simulink model "IEEE33_2018"  (R2018b)
settings: Solver=VariableStepAuto  StartTime=0.0  StopTime=0.04  RelTol=1e-3
undefined symbols (not defined in the file or in its folder): D11, Delta
libraries: powerlib x134
settings Model: Creator=zyx  LastModifiedBy=zyx53
settings DataIOCC: ReturnWorkspaceOutputs=on
settings DebuggingCC: UnconnectedInputMsg=none  UnconnectedOutputMsg=none  UnconnectedLineMsg=none
settings ModelReferenceCC: EnableRefExpFcnMdlSchedulingChecks=off
settings RTWCC: Description=Generic Real-Time Target

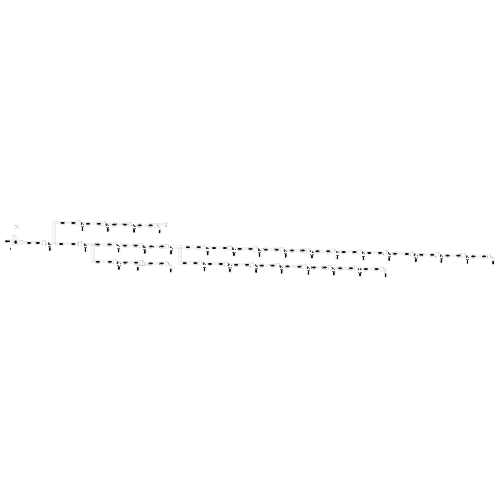
[thumbnail: Simulink's stored preview of the top-level diagram]
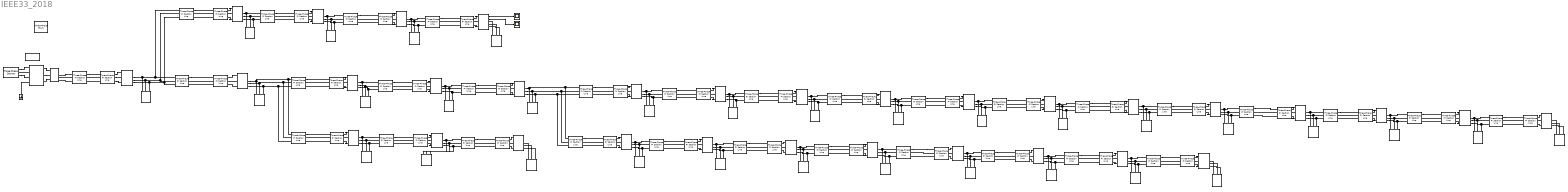
== system IEEE33_2018 ==
  Ground : powerlib/Elements/Ground  LConnTagsString=a
  Node1 : powerlib/Elements/Three-Phase Series RLC Load  LConnTagsString=A|B|C  Configuration=Y (grounded)  NominalVoltage=10.5e3  Vabc=[1e3 1e3 1e3]  Vabcp=[1e3 1e3 1e3]  NominalFrequency=50  UnbalancedPower=off  ActivePower=1636286.9  InductivePower=425428.22  CapacitivePower=0  Pabc=[10e3 9e3 11e3]  QLabc=[100 90 110]  QCabc=[100 90 110]  Pabcp=[10e3 9e3 11e3]  QLabcp=[100 90 110]  QCabcp=[100 90 110]  Measurements=None  LoadType=constant Z
  Node10 : powerlib/Elements/Three-Phase Series RLC Load  LConnTagsString=A|B|C  Configuration=Y (grounded)  NominalVoltage=10.5e3  Vabc=[1e3 1e3 1e3]  Vabcp=[1e3 1e3 1e3]  NominalFrequency=50  UnbalancedPower=off  ActivePower=1452178.34  InductivePower=456782.16  CapacitivePower=0  Pabc=[10e3 9e3 11e3]  QLabc=[100 90 110]  QCabc=[100 90 110]  Pabcp=[10e3 9e3 11e3]  QLabcp=[100 90 110]  QCabcp=[100 90 110]  Measurements=None  LoadType=constant Z
  Node11 : powerlib/Elements/Three-Phase Series RLC Load  LConnTagsString=A|B|C  Configuration=Y (grounded)  NominalVoltage=10.5e3  Vabc=[1e3 1e3 1e3]  Vabcp=[1e3 1e3 1e3]  NominalFrequency=50  UnbalancedPower=off  ActivePower=1330341.72  InductivePower=405395.01  CapacitivePower=0  Pabc=[10e3 9e3 11e3]  QLabc=[100 90 110]  QCabc=[100 90 110]  Pabcp=[10e3 9e3 11e3]  QLabcp=[100 90 110]  QCabcp=[100 90 110]  Measurements=None  LoadType=constant Z
  Node12 : powerlib/Elements/Three-Phase Series RLC Load  LConnTagsString=A|B|C  Configuration=Y (grounded)  NominalVoltage=10.5e3  Vabc=[1e3 1e3 1e3]  Vabcp=[1e3 1e3 1e3]  NominalFrequency=50  UnbalancedPower=off  ActivePower=1512319.02  InductivePower=477916.72  CapacitivePower=0  Pabc=[10e3 9e3 11e3]  QLabc=[100 90 110]  QCabc=[100 90 110]  Pabcp=[10e3 9e3 11e3]  QLabcp=[100 90 110]  QCabcp=[100 90 110]  Measurements=None  LoadType=constant Z
  Node13 : powerlib/Elements/Three-Phase Series RLC Load  LConnTagsString=A|B|C  Configuration=Y (grounded)  NominalVoltage=10.5e3  Vabc=[1e3 1e3 1e3]  Vabcp=[1e3 1e3 1e3]  NominalFrequency=50  UnbalancedPower=off  ActivePower=1673604.27  InductivePower=412990.62  CapacitivePower=0  Pabc=[10e3 9e3 11e3]  QLabc=[100 90 110]  QCabc=[100 90 110]  Pabcp=[10e3 9e3 11e3]  QLabcp=[100 90 110]  QCabcp=[100 90 110]  Measurements=None  LoadType=constant Z
  Node14 : powerlib/Elements/Three-Phase Series RLC Load  LConnTagsString=A|B|C  Configuration=Y (grounded)  NominalVoltage=10.5e3  Vabc=[1e3 1e3 1e3]  Vabcp=[1e3 1e3 1e3]  NominalFrequency=50  UnbalancedPower=off  ActivePower=1527529.46  InductivePower=446939.06  CapacitivePower=0  Pabc=[10e3 9e3 11e3]  QLabc=[100 90 110]  QCabc=[100 90 110]  Pabcp=[10e3 9e3 11e3]  QLabcp=[100 90 110]  QCabcp=[100 90 110]  Measurements=None  LoadType=constant Z
  Node15 : powerlib/Elements/Three-Phase Series RLC Load  LConnTagsString=A|B|C  Configuration=Y (grounded)  NominalVoltage=10.5e3  Vabc=[1e3 1e3 1e3]  Vabcp=[1e3 1e3 1e3]  NominalFrequency=50  UnbalancedPower=off  ActivePower=1304760.83  InductivePower=433712.26  CapacitivePower=0  Pabc=[10e3 9e3 11e3]  QLabc=[100 90 110]  QCabc=[100 90 110]  Pabcp=[10e3 9e3 11e3]  QLabcp=[100 90 110]  QCabcp=[100 90 110]  Measurements=None  LoadType=constant Z
  Node16 : powerlib/Elements/Three-Phase Series RLC Load  LConnTagsString=A|B|C  Configuration=Y (grounded)  NominalVoltage=10.5e3  Vabc=[1e3 1e3 1e3]  Vabcp=[1e3 1e3 1e3]  NominalFrequency=50  UnbalancedPower=off  ActivePower=1364872.92  InductivePower=479428.45  CapacitivePower=0  Pabc=[10e3 9e3 11e3]  QLabc=[100 90 110]  QCabc=[100 90 110]  Pabcp=[10e3 9e3 11e3]  QLabcp=[100 90 110]  QCabcp=[100 90 110]  Measurements=None  LoadType=constant Z
  Node17 : powerlib/Elements/Three-Phase Series RLC Load  LConnTagsString=A|B|C  Configuration=Y (grounded)  NominalVoltage=10.5e3  Vabc=[1e3 1e3 1e3]  Vabcp=[1e3 1e3 1e3]  NominalFrequency=50  UnbalancedPower=off  ActivePower=1424486.02  InductivePower=452853.31  CapacitivePower=0  Pabc=[10e3 9e3 11e3]  QLabc=[100 90 110]  QCabc=[100 90 110]  Pabcp=[10e3 9e3 11e3]  QLabcp=[100 90 110]  QCabcp=[100 90 110]  Measurements=None  LoadType=constant Z
  Node18 : powerlib/Elements/Three-Phase Series RLC Load  LConnTagsString=A|B|C  Configuration=Y (grounded)  NominalVoltage=10.5e3  Vabc=[1e3 1e3 1e3]  Vabcp=[1e3 1e3 1e3]  NominalFrequency=50  UnbalancedPower=off  ActivePower=1366259.49  InductivePower=460198.19  CapacitivePower=0  Pabc=[10e3 9e3 11e3]  QLabc=[100 90 110]  QCabc=[100 90 110]  Pabcp=[10e3 9e3 11e3]  QLabcp=[100 90 110]  QCabcp=[100 90 110]  Measurements=None  LoadType=constant Z
  Node19 : powerlib/Elements/Three-Phase Series RLC Load  LConnTagsString=A|B|C  Configuration=Y (grounded)  NominalVoltage=10.5e3  Vabc=[1e3 1e3 1e3]  Vabcp=[1e3 1e3 1e3]  NominalFrequency=50  UnbalancedPower=off  ActivePower=1405188.51  InductivePower=465407.91  CapacitivePower=0  Pabc=[10e3 9e3 11e3]  QLabc=[100 90 110]  QCabc=[100 90 110]  Pabcp=[10e3 9e3 11e3]  QLabcp=[100 90 110]  QCabcp=[100 90 110]  Measurements=None  LoadType=constant Z
  Node2 : powerlib/Elements/Three-Phase Series RLC Load  LConnTagsString=A|B|C  Configuration=Y (grounded)  NominalVoltage=10.5e3  Vabc=[1e3 1e3 1e3]  Vabcp=[1e3 1e3 1e3]  NominalFrequency=50  UnbalancedPower=off  ActivePower=1625713.93  InductivePower=424352.5  CapacitivePower=0  Pabc=[10e3 9e3 11e3]  QLabc=[100 90 110]  QCabc=[100 90 110]  Pabcp=[10e3 9e3 11e3]  QLabcp=[100 90 110]  QCabcp=[100 90 110]  Measurements=None  LoadType=constant Z
  Node20 : powerlib/Elements/Three-Phase Series RLC Load  LConnTagsString=A|B|C  Configuration=Y (grounded)  NominalVoltage=10.5e3  Vabc=[1e3 1e3 1e3]  Vabcp=[1e3 1e3 1e3]  NominalFrequency=50  UnbalancedPower=off  ActivePower=1575685.8  InductivePower=474815.16  CapacitivePower=0  Pabc=[10e3 9e3 11e3]  QLabc=[100 90 110]  QCabc=[100 90 110]  Pabcp=[10e3 9e3 11e3]  QLabcp=[100 90 110]  QCabcp=[100 90 110]  Measurements=None  LoadType=constant Z
  Node21 : powerlib/Elements/Three-Phase Series RLC Load  LConnTagsString=A|B|C  Configuration=Y (grounded)  NominalVoltage=10.5e3  Vabc=[1e3 1e3 1e3]  Vabcp=[1e3 1e3 1e3]  NominalFrequency=50  UnbalancedPower=off  ActivePower=1480216.64  InductivePower=408382.14  CapacitivePower=0  Pabc=[10e3 9e3 11e3]  QLabc=[100 90 110]  QCabc=[100 90 110]  Pabcp=[10e3 9e3 11e3]  QLabcp=[100 90 110]  QCabcp=[100 90 110]  Measurements=None  LoadType=constant Z
  Node22 : powerlib/Elements/Three-Phase Series RLC Load  LConnTagsString=A|B|C  Configuration=Y (grounded)  NominalVoltage=10.5e3  Vabc=[1e3 1e3 1e3]  Vabcp=[1e3 1e3 1e3]  NominalFrequency=50  UnbalancedPower=off  ActivePower=1391590.79  InductivePower=491333.74  CapacitivePower=0  Pabc=[10e3 9e3 11e3]  QLabc=[100 90 110]  QCabc=[100 90 110]  Pabcp=[10e3 9e3 11e3]  QLabcp=[100 90 110]  QCabcp=[100 90 110]  Measurements=None  LoadType=constant Z
  Node23 : powerlib/Elements/Three-Phase Series RLC Load  LConnTagsString=A|B|C  Configuration=Y (grounded)  NominalVoltage=10.5e3  Vabc=[1e3 1e3 1e3]  Vabcp=[1e3 1e3 1e3]  NominalFrequency=50  UnbalancedPower=off  ActivePower=1360951.21  InductivePower=482581.7  CapacitivePower=0  Pabc=[10e3 9e3 11e3]  QLabc=[100 90 110]  QCabc=[100 90 110]  Pabcp=[10e3 9e3 11e3]  QLabcp=[100 90 110]  QCabcp=[100 90 110]  Measurements=None  LoadType=constant Z
  Node24 : powerlib/Elements/Three-Phase Series RLC Load  LConnTagsString=A|B|C  Configuration=Y (grounded)  NominalVoltage=10.5e3  Vabc=[1e3 1e3 1e3]  Vabcp=[1e3 1e3 1e3]  NominalFrequency=50  UnbalancedPower=off  ActivePower=1515336.97  InductivePower=499613.47  CapacitivePower=0  Pabc=[10e3 9e3 11e3]  QLabc=[100 90 110]  QCabc=[100 90 110]  Pabcp=[10e3 9e3 11e3]  QLabcp=[100 90 110]  QCabcp=[100 90 110]  Measurements=None  LoadType=constant Z
  Node25 : powerlib/Elements/Three-Phase Series RLC Load  LConnTagsString=A|B|C  Configuration=Y (grounded)  NominalVoltage=10.5e3  Vabc=[1e3 1e3 1e3]  Vabcp=[1e3 1e3 1e3]  NominalFrequency=50  UnbalancedPower=off  ActivePower=1331270.21  InductivePower=444267.83  CapacitivePower=0  Pabc=[10e3 9e3 11e3]  QLabc=[100 90 110]  QCabc=[100 90 110]  Pabcp=[10e3 9e3 11e3]  QLabcp=[100 90 110]  QCabcp=[100 90 110]  Measurements=None  LoadType=constant Z
  Node26 : powerlib/Elements/Three-Phase Series RLC Load  LConnTagsString=A|B|C  Configuration=Y (grounded)  NominalVoltage=10.5e3  Vabc=[1e3 1e3 1e3]  Vabcp=[1e3 1e3 1e3]  NominalFrequency=50  UnbalancedPower=off  ActivePower=1342661.11  InductivePower=496189.81  CapacitivePower=0  Pabc=[10e3 9e3 11e3]  QLabc=[100 90 110]  QCabc=[100 90 110]  Pabcp=[10e3 9e3 11e3]  QLabcp=[100 90 110]  QCabcp=[100 90 110]  Measurements=None  LoadType=constant Z
  Node27 : powerlib/Elements/Three-Phase Series RLC Load  LConnTagsString=A|B|C  Configuration=Y (grounded)  NominalVoltage=10.5e3  Vabc=[1e3 1e3 1e3]  Vabcp=[1e3 1e3 1e3]  NominalFrequency=50  UnbalancedPower=off  ActivePower=1301853.69  InductivePower=477491.05  CapacitivePower=0  Pabc=[10e3 9e3 11e3]  QLabc=[100 90 110]  QCabc=[100 90 110]  Pabcp=[10e3 9e3 11e3]  QLabcp=[100 90 110]  QCabcp=[100 90 110]  Measurements=None  LoadType=constant Z
  Node28 : powerlib/Elements/Three-Phase Series RLC Load  LConnTagsString=A|B|C  Configuration=Y (grounded)  NominalVoltage=10.5e3  Vabc=[1e3 1e3 1e3]  Vabcp=[1e3 1e3 1e3]  NominalFrequency=50  UnbalancedPower=off  ActivePower=1626921.29  InductivePower=486869.47  CapacitivePower=0  Pabc=[10e3 9e3 11e3]  QLabc=[100 90 110]  QCabc=[100 90 110]  Pabcp=[10e3 9e3 11e3]  QLabcp=[100 90 110]  QCabcp=[100 90 110]  Measurements=None  LoadType=constant Z
  Node29 : powerlib/Elements/Three-Phase Series RLC Load  LConnTagsString=A|B|C  Configuration=Y (grounded)  NominalVoltage=10.5e3  Vabc=[1e3 1e3 1e3]  Vabcp=[1e3 1e3 1e3]  NominalFrequency=50  UnbalancedPower=off  ActivePower=1333774.34  InductivePower=439978.26  CapacitivePower=0  Pabc=[10e3 9e3 11e3]  QLabc=[100 90 110]  QCabc=[100 90 110]  Pabcp=[10e3 9e3 11e3]  QLabcp=[100 90 110]  QCabcp=[100 90 110]  Measurements=None  LoadType=constant Z
  Node3 : powerlib/Elements/Three-Phase Series RLC Load  LConnTagsString=A|B|C  Configuration=Y (grounded)  NominalVoltage=10.5e3  Vabc=[1e3 1e3 1e3]  Vabcp=[1e3 1e3 1e3]  NominalFrequency=50  UnbalancedPower=off  ActivePower=1671705.45  InductivePower=434998.38  CapacitivePower=0  Pabc=[10e3 9e3 11e3]  QLabc=[100 90 110]  QCabc=[100 90 110]  Pabcp=[10e3 9e3 11e3]  QLabcp=[100 90 110]  QCabcp=[100 90 110]  Measurements=None  LoadType=constant Z
  Node30 : powerlib/Elements/Three-Phase Series RLC Load  LConnTagsString=A|B|C  Configuration=Y (grounded)  NominalVoltage=10.5e3  Vabc=[1e3 1e3 1e3]  Vabcp=[1e3 1e3 1e3]  NominalFrequency=50  UnbalancedPower=off  ActivePower=1403948.16  InductivePower=480006.85  CapacitivePower=0  Pabc=[10e3 9e3 11e3]  QLabc=[100 90 110]  QCabc=[100 90 110]  Pabcp=[10e3 9e3 11e3]  QLabcp=[100 90 110]  QCabcp=[100 90 110]  Measurements=None  LoadType=constant Z
  Node31 : powerlib/Elements/Three-Phase Series RLC Load  LConnTagsString=A|B|C  Configuration=Y (grounded)  NominalVoltage=10.5e3  Vabc=[1e3 1e3 1e3]  Vabcp=[1e3 1e3 1e3]  NominalFrequency=50  UnbalancedPower=off  ActivePower=1472565.53  InductivePower=491064.76  CapacitivePower=0  Pabc=[10e3 9e3 11e3]  QLabc=[100 90 110]  QCabc=[100 90 110]  Pabcp=[10e3 9e3 11e3]  QLabcp=[100 90 110]  QCabcp=[100 90 110]  Measurements=None  LoadType=constant Z
  Node32 : powerlib/Elements/Three-Phase Series RLC Load  LConnTagsString=A|B|C  Configuration=Y (grounded)  NominalVoltage=10.5e3  Vabc=[1e3 1e3 1e3]  Vabcp=[1e3 1e3 1e3]  NominalFrequency=50  UnbalancedPower=off  ActivePower=1372738.81  InductivePower=426380.29  CapacitivePower=0  Pabc=[10e3 9e3 11e3]  QLabc=[100 90 110]  QCabc=[100 90 110]  Pabcp=[10e3 9e3 11e3]  QLabcp=[100 90 110]  QCabcp=[100 90 110]  Measurements=None  LoadType=constant Z
  Node4 : powerlib/Elements/Three-Phase Series RLC Load  LConnTagsString=A|B|C  Configuration=Y (grounded)  NominalVoltage=10.5e3  Vabc=[1e3 1e3 1e3]  Vabcp=[1e3 1e3 1e3]  NominalFrequency=50  UnbalancedPower=off  ActivePower=1378638.1  InductivePower=425108.39  CapacitivePower=0  Pabc=[10e3 9e3 11e3]  QLabc=[100 90 110]  QCabc=[100 90 110]  Pabcp=[10e3 9e3 11e3]  QLabcp=[100 90 110]  QCabcp=[100 90 110]  Measurements=None  LoadType=constant Z
  Node5 : powerlib/Elements/Three-Phase Series RLC Load  LConnTagsString=A|B|C  Configuration=Y (grounded)  NominalVoltage=10.5e3  Vabc=[1e3 1e3 1e3]  Vabcp=[1e3 1e3 1e3]  NominalFrequency=50  UnbalancedPower=off  ActivePower=1546417.87  InductivePower=447328.88  CapacitivePower=0  Pabc=[10e3 9e3 11e3]  QLabc=[100 90 110]  QCabc=[100 90 110]  Pabcp=[10e3 9e3 11e3]  QLabcp=[100 90 110]  QCabcp=[100 90 110]  Measurements=None  LoadType=constant Z
  Node6 : powerlib/Elements/Three-Phase Series RLC Load  LConnTagsString=A|B|C  Configuration=Y (grounded)  NominalVoltage=10.5e3  Vabc=[1e3 1e3 1e3]  Vabcp=[1e3 1e3 1e3]  NominalFrequency=50  UnbalancedPower=off  ActivePower=1440663.8  InductivePower=483082.86  CapacitivePower=0  Pabc=[10e3 9e3 11e3]  QLabc=[100 90 110]  QCabc=[100 90 110]  Pabcp=[10e3 9e3 11e3]  QLabcp=[100 90 110]  QCabcp=[100 90 110]  Measurements=None  LoadType=constant Z
  Node7 : powerlib/Elements/Three-Phase Series RLC Load  LConnTagsString=A|B|C  Configuration=Y (grounded)  NominalVoltage=10.5e3  Vabc=[1e3 1e3 1e3]  Vabcp=[1e3 1e3 1e3]  NominalFrequency=50  UnbalancedPower=off  ActivePower=1534105.64  InductivePower=454972.36  CapacitivePower=0  Pabc=[10e3 9e3 11e3]  QLabc=[100 90 110]  QCabc=[100 90 110]  Pabcp=[10e3 9e3 11e3]  QLabcp=[100 90 110]  QCabcp=[100 90 110]  Measurements=None  LoadType=constant Z
  Node8 : powerlib/Elements/Three-Phase Series RLC Load  LConnTagsString=A|B|C  Configuration=Y (grounded)  NominalVoltage=10.5e3  Vabc=[1e3 1e3 1e3]  Vabcp=[1e3 1e3 1e3]  NominalFrequency=50  UnbalancedPower=off  ActivePower=1666877.47  InductivePower=428583.9  CapacitivePower=0  Pabc=[10e3 9e3 11e3]  QLabc=[100 90 110]  QCabc=[100 90 110]  Pabcp=[10e3 9e3 11e3]  QLabcp=[100 90 110]  QCabcp=[100 90 110]  Measurements=None  LoadType=constant Z
  Node9 : powerlib/Elements/Three-Phase Series RLC Load  LConnTagsString=A|B|C  Configuration=Y (grounded)  NominalVoltage=10.5e3  Vabc=[1e3 1e3 1e3]  Vabcp=[1e3 1e3 1e3]  NominalFrequency=50  UnbalancedPower=off  ActivePower=1602880.09  InductivePower=475372.91  CapacitivePower=0  Pabc=[10e3 9e3 11e3]  QLabc=[100 90 110]  QCabc=[100 90 110]  Pabcp=[10e3 9e3 11e3]  QLabcp=[100 90 110]  QCabcp=[100 90 110]  Measurements=None  LoadType=constant Z
  Scope : Scope
  Scope1 : Scope
  Three-Phase Transformer (Two Windings) : powerlib/Elements/Three-Phase Transformer (Two Windings)  Winding1Connection=Yn  Winding2Connection=Delta (D11)  CoreType=Three single-phase transformers  SetSaturation=off  Hysteresis=off  DataFile='hysteresis'  SetInitialFlux=off  Measurements=None  UNITS=pu  NominalPower=[ 200e6 , 50 ]  Winding1=[ 110e3 , 0.002 , 0.08 ]  Winding2=[ 10.5e3 , 0.002 , 0.08 ]  Rm=500  Lm=500  L0=0.5  Saturation=[ 0,0 ; 0.0024,1.2 ; 1.0,1.52 ]  InitialFluxes=[ 0.8 , -0.8 , 0.7 ]  BreakLoop=off  DiscreteSolver=Trapezoidal iterative  DataType=off  TransfoNumber=1
  Three-Phase V-I Measurement{,1..32} (33 alike) : powerlib/Measurements/Three-Phase V-I Measurement  VoltageMeasurement=phase-to-ground  SetLabelV=off  LabelV=Vabc  Vpu=off  VpuLL=off  CurrentMeasurement=yes  SetLabelI=off  LabelI=Iabc  Ipu=off  Pbase=100e6  Vbase=500e3  OutputType=Complex  PhasorSimulation=off  PSBequivalent=0
  Three-Phase Fault : powerlib/Elements/Three-Phase Fault  InitialStates=0  FaultA=on  FaultB=off  FaultC=off  GroundFault=on  SwitchTimes=[0 ]  External=off  SwitchStatus=NaN  FaultResistance=0.001  GroundResistance=0.01  SnubberResistance=1e6  SnubberCapacitance=inf  Measurements=None
  Three-Phase Source : powerlib/Electrical Sources/Three-Phase Source  InternalConnection=Yg  VoltagePhases=off  Voltage=110e3  PhaseAngle=0  Voltage_phases=[25e3 25e3 25e3]/sqrt(3)  PhaseAngles_phases=[0 -120 +120]  Frequency=50  NonIdealSource=on  SpecifyImpedance=off  Resistance=5.74  Inductance=0.0452  ShortCircuitLevel=100e6  BaseVoltage=110e3/(3^0.5)  XRratio=7  BusType=swing  Pref=10e3  Qref=0  Prefabc=[10e3, 10e3, 10e3]  Qrefabc=[0, 0, 0]  Qmin=-inf  Qmax=inf
  line10_1 : powerlib/Elements/Three-Phase PI Section Line  LConnTagsString=a|b|c  RConnTagsString=A|B|C  Length=0.1  Frequency=60  Resistances=[ 0.01273 0.3864]  Inductances="[ 0.9337e-3  4.1264e-3]"  Capacitances=[12.74e-9 7.751e-9]
  line10_2 : powerlib/Elements/Three-Phase PI Section Line  LConnTagsString=a|b|c  RConnTagsString=A|B|C  Length=0.9  Frequency=60  Resistances=[ 0.01273 0.3864]  Inductances="[ 0.9337e-3  4.1264e-3]"  Capacitances=[12.74e-9 7.751e-9]
  line11_1 : powerlib/Elements/Three-Phase PI Section Line  LConnTagsString=a|b|c  RConnTagsString=A|B|C  Length=0.1  Frequency=60  Resistances=[ 0.01273 0.3864]  Inductances="[ 0.9337e-3  4.1264e-3]"  Capacitances=[12.74e-9 7.751e-9]
  line11_2 : powerlib/Elements/Three-Phase PI Section Line  LConnTagsString=a|b|c  RConnTagsString=A|B|C  Length=0.9  Frequency=60  Resistances=[ 0.01273 0.3864]  Inductances="[ 0.9337e-3  4.1264e-3]"  Capacitances=[12.74e-9 7.751e-9]
  line12_1 : powerlib/Elements/Three-Phase PI Section Line  LConnTagsString=a|b|c  RConnTagsString=A|B|C  Length=0.1  Frequency=60  Resistances=[ 0.01273 0.3864]  Inductances="[ 0.9337e-3  4.1264e-3]"  Capacitances=[12.74e-9 7.751e-9]
  line12_2 : powerlib/Elements/Three-Phase PI Section Line  LConnTagsString=a|b|c  RConnTagsString=A|B|C  Length=0.9  Frequency=60  Resistances=[ 0.01273 0.3864]  Inductances="[ 0.9337e-3  4.1264e-3]"  Capacitances=[12.74e-9 7.751e-9]
  line13_1 : powerlib/Elements/Three-Phase PI Section Line  LConnTagsString=a|b|c  RConnTagsString=A|B|C  Length=0.1  Frequency=60  Resistances=[ 0.01273 0.3864]  Inductances="[ 0.9337e-3  4.1264e-3]"  Capacitances=[12.74e-9 7.751e-9]
  line13_2 : powerlib/Elements/Three-Phase PI Section Line  LConnTagsString=a|b|c  RConnTagsString=A|B|C  Length=0.9  Frequency=60  Resistances=[ 0.01273 0.3864]  Inductances="[ 0.9337e-3  4.1264e-3]"  Capacitances=[12.74e-9 7.751e-9]
  line14_1 : powerlib/Elements/Three-Phase PI Section Line  LConnTagsString=a|b|c  RConnTagsString=A|B|C  Length=0.1  Frequency=60  Resistances=[ 0.01273 0.3864]  Inductances="[ 0.9337e-3  4.1264e-3]"  Capacitances=[12.74e-9 7.751e-9]
  line14_2 : powerlib/Elements/Three-Phase PI Section Line  LConnTagsString=a|b|c  RConnTagsString=A|B|C  Length=0.9  Frequency=60  Resistances=[ 0.01273 0.3864]  Inductances="[ 0.9337e-3  4.1264e-3]"  Capacitances=[12.74e-9 7.751e-9]
  line15_1 : powerlib/Elements/Three-Phase PI Section Line  LConnTagsString=a|b|c  RConnTagsString=A|B|C  Length=0.1  Frequency=60  Resistances=[ 0.01273 0.3864]  Inductances="[ 0.9337e-3  4.1264e-3]"  Capacitances=[12.74e-9 7.751e-9]
  line15_2 : powerlib/Elements/Three-Phase PI Section Line  LConnTagsString=a|b|c  RConnTagsString=A|B|C  Length=0.9  Frequency=60  Resistances=[ 0.01273 0.3864]  Inductances="[ 0.9337e-3  4.1264e-3]"  Capacitances=[12.74e-9 7.751e-9]
  line16_1 : powerlib/Elements/Three-Phase PI Section Line  LConnTagsString=a|b|c  RConnTagsString=A|B|C  Length=0.1  Frequency=60  Resistances=[ 0.01273 0.3864]  Inductances="[ 0.9337e-3  4.1264e-3]"  Capacitances=[12.74e-9 7.751e-9]
  line16_2 : powerlib/Elements/Three-Phase PI Section Line  LConnTagsString=a|b|c  RConnTagsString=A|B|C  Length=0.9  Frequency=60  Resistances=[ 0.01273 0.3864]  Inductances="[ 0.9337e-3  4.1264e-3]"  Capacitances=[12.74e-9 7.751e-9]
  line17_1 : powerlib/Elements/Three-Phase PI Section Line  LConnTagsString=a|b|c  RConnTagsString=A|B|C  Length=0.1  Frequency=60  Resistances=[ 0.01273 0.3864]  Inductances="[ 0.9337e-3  4.1264e-3]"  Capacitances=[12.74e-9 7.751e-9]
  line17_2 : powerlib/Elements/Three-Phase PI Section Line  LConnTagsString=a|b|c  RConnTagsString=A|B|C  Length=0.9  Frequency=60  Resistances=[ 0.01273 0.3864]  Inductances="[ 0.9337e-3  4.1264e-3]"  Capacitances=[12.74e-9 7.751e-9]
  line18_1 : powerlib/Elements/Three-Phase PI Section Line  LConnTagsString=a|b|c  RConnTagsString=A|B|C  Length=0.1  Frequency=60  Resistances=[ 0.01273 0.3864]  Inductances="[ 0.9337e-3  4.1264e-3]"  Capacitances=[12.74e-9 7.751e-9]
  line18_2 : powerlib/Elements/Three-Phase PI Section Line  LConnTagsString=a|b|c  RConnTagsString=A|B|C  Length=0.9  Frequency=60  Resistances=[ 0.01273 0.3864]  Inductances="[ 0.9337e-3  4.1264e-3]"  Capacitances=[12.74e-9 7.751e-9]
  line19_1 : powerlib/Elements/Three-Phase PI Section Line  LConnTagsString=a|b|c  RConnTagsString=A|B|C  Length=0.1  Frequency=60  Resistances=[ 0.01273 0.3864]  Inductances="[ 0.9337e-3  4.1264e-3]"  Capacitances=[12.74e-9 7.751e-9]
  line19_2 : powerlib/Elements/Three-Phase PI Section Line  LConnTagsString=a|b|c  RConnTagsString=A|B|C  Length=0.9  Frequency=60  Resistances=[ 0.01273 0.3864]  Inductances="[ 0.9337e-3  4.1264e-3]"  Capacitances=[12.74e-9 7.751e-9]
  line1_1 : powerlib/Elements/Three-Phase PI Section Line  LConnTagsString=a|b|c  RConnTagsString=A|B|C  Length=0.1  Frequency=60  Resistances=[ 0.01273 0.3864]  Inductances="[ 0.9337e-3  4.1264e-3]"  Capacitances=[12.74e-9 7.751e-9]
  line1_2 : powerlib/Elements/Three-Phase PI Section Line  LConnTagsString=a|b|c  RConnTagsString=A|B|C  Length=0.9  Frequency=60  Resistances=[ 0.01273 0.3864]  Inductances="[ 0.9337e-3  4.1264e-3]"  Capacitances=[12.74e-9 7.751e-9]
  line20_1 : powerlib/Elements/Three-Phase PI Section Line  LConnTagsString=a|b|c  RConnTagsString=A|B|C  Length=0.1  Frequency=60  Resistances=[ 0.01273 0.3864]  Inductances="[ 0.9337e-3  4.1264e-3]"  Capacitances=[12.74e-9 7.751e-9]
  line20_2 : powerlib/Elements/Three-Phase PI Section Line  LConnTagsString=a|b|c  RConnTagsString=A|B|C  Length=0.9  Frequency=60  Resistances=[ 0.01273 0.3864]  Inductances="[ 0.9337e-3  4.1264e-3]"  Capacitances=[12.74e-9 7.751e-9]
  line21_1 : powerlib/Elements/Three-Phase PI Section Line  LConnTagsString=a|b|c  RConnTagsString=A|B|C  Length=0.1  Frequency=60  Resistances=[ 0.01273 0.3864]  Inductances="[ 0.9337e-3  4.1264e-3]"  Capacitances=[12.74e-9 7.751e-9]
  line21_2 : powerlib/Elements/Three-Phase PI Section Line  LConnTagsString=a|b|c  RConnTagsString=A|B|C  Length=0.9  Frequency=60  Resistances=[ 0.01273 0.3864]  Inductances="[ 0.9337e-3  4.1264e-3]"  Capacitances=[12.74e-9 7.751e-9]
  line22_1 : powerlib/Elements/Three-Phase PI Section Line  LConnTagsString=a|b|c  RConnTagsString=A|B|C  Length=0.1  Frequency=60  Resistances=[ 0.01273 0.3864]  Inductances="[ 0.9337e-3  4.1264e-3]"  Capacitances=[12.74e-9 7.751e-9]
  line22_2 : powerlib/Elements/Three-Phase PI Section Line  LConnTagsString=a|b|c  RConnTagsString=A|B|C  Length=0.9  Frequency=60  Resistances=[ 0.01273 0.3864]  Inductances="[ 0.9337e-3  4.1264e-3]"  Capacitances=[12.74e-9 7.751e-9]
  line23_1 : powerlib/Elements/Three-Phase PI Section Line  LConnTagsString=a|b|c  RConnTagsString=A|B|C  Length=0.1  Frequency=60  Resistances=[ 0.01273 0.3864]  Inductances="[ 0.9337e-3  4.1264e-3]"  Capacitances=[12.74e-9 7.751e-9]
  line23_2 : powerlib/Elements/Three-Phase PI Section Line  LConnTagsString=a|b|c  RConnTagsString=A|B|C  Length=0.9  Frequency=60  Resistances=[ 0.01273 0.3864]  Inductances="[ 0.9337e-3  4.1264e-3]"  Capacitances=[12.74e-9 7.751e-9]
  line24_1 : powerlib/Elements/Three-Phase PI Section Line  LConnTagsString=a|b|c  RConnTagsString=A|B|C  Length=0.1  Frequency=60  Resistances=[ 0.01273 0.3864]  Inductances="[ 0.9337e-3  4.1264e-3]"  Capacitances=[12.74e-9 7.751e-9]
  line24_2 : powerlib/Elements/Three-Phase PI Section Line  LConnTagsString=a|b|c  RConnTagsString=A|B|C  Length=0.9  Frequency=60  Resistances=[ 0.01273 0.3864]  Inductances="[ 0.9337e-3  4.1264e-3]"  Capacitances=[12.74e-9 7.751e-9]
  line25_1 : powerlib/Elements/Three-Phase PI Section Line  LConnTagsString=a|b|c  RConnTagsString=A|B|C  Length=0.1  Frequency=60  Resistances=[ 0.01273 0.3864]  Inductances="[ 0.9337e-3  4.1264e-3]"  Capacitances=[12.74e-9 7.751e-9]
  line25_2 : powerlib/Elements/Three-Phase PI Section Line  LConnTagsString=a|b|c  RConnTagsString=A|B|C  Length=0.9  Frequency=60  Resistances=[ 0.01273 0.3864]  Inductances="[ 0.9337e-3  4.1264e-3]"  Capacitances=[12.74e-9 7.751e-9]
  line26_1 : powerlib/Elements/Three-Phase PI Section Line  LConnTagsString=a|b|c  RConnTagsString=A|B|C  Length=0.1  Frequency=60  Resistances=[ 0.01273 0.3864]  Inductances="[ 0.9337e-3  4.1264e-3]"  Capacitances=[12.74e-9 7.751e-9]
  line26_2 : powerlib/Elements/Three-Phase PI Section Line  LConnTagsString=a|b|c  RConnTagsString=A|B|C  Length=0.9  Frequency=60  Resistances=[ 0.01273 0.3864]  Inductances="[ 0.9337e-3  4.1264e-3]"  Capacitances=[12.74e-9 7.751e-9]
  line27_1 : powerlib/Elements/Three-Phase PI Section Line  LConnTagsString=a|b|c  RConnTagsString=A|B|C  Length=0.1  Frequency=60  Resistances=[ 0.01273 0.3864]  Inductances="[ 0.9337e-3  4.1264e-3]"  Capacitances=[12.74e-9 7.751e-9]
  line27_2 : powerlib/Elements/Three-Phase PI Section Line  LConnTagsString=a|b|c  RConnTagsString=A|B|C  Length=0.9  Frequency=60  Resistances=[ 0.01273 0.3864]  Inductances="[ 0.9337e-3  4.1264e-3]"  Capacitances=[12.74e-9 7.751e-9]
  line28_1 : powerlib/Elements/Three-Phase PI Section Line  LConnTagsString=a|b|c  RConnTagsString=A|B|C  Length=0.1  Frequency=60  Resistances=[ 0.01273 0.3864]  Inductances="[ 0.9337e-3  4.1264e-3]"  Capacitances=[12.74e-9 7.751e-9]
  line28_2 : powerlib/Elements/Three-Phase PI Section Line  LConnTagsString=a|b|c  RConnTagsString=A|B|C  Length=0.9  Frequency=60  Resistances=[ 0.01273 0.3864]  Inductances="[ 0.9337e-3  4.1264e-3]"  Capacitances=[12.74e-9 7.751e-9]
  line29_1 : powerlib/Elements/Three-Phase PI Section Line  LConnTagsString=a|b|c  RConnTagsString=A|B|C  Length=0.1  Frequency=60  Resistances=[ 0.01273 0.3864]  Inductances="[ 0.9337e-3  4.1264e-3]"  Capacitances=[12.74e-9 7.751e-9]
  line29_2 : powerlib/Elements/Three-Phase PI Section Line  LConnTagsString=a|b|c  RConnTagsString=A|B|C  Length=0.9  Frequency=60  Resistances=[ 0.01273 0.3864]  Inductances="[ 0.9337e-3  4.1264e-3]"  Capacitances=[12.74e-9 7.751e-9]
  line2_1 : powerlib/Elements/Three-Phase PI Section Line  LConnTagsString=a|b|c  RConnTagsString=A|B|C  Length=0.1  Frequency=60  Resistances=[ 0.01273 0.3864]  Inductances="[ 0.9337e-3  4.1264e-3]"  Capacitances=[12.74e-9 7.751e-9]
  line2_2 : powerlib/Elements/Three-Phase PI Section Line  LConnTagsString=a|b|c  RConnTagsString=A|B|C  Length=0.9  Frequency=60  Resistances=[ 0.01273 0.3864]  Inductances="[ 0.9337e-3  4.1264e-3]"  Capacitances=[12.74e-9 7.751e-9]
  line30_1 : powerlib/Elements/Three-Phase PI Section Line  LConnTagsString=a|b|c  RConnTagsString=A|B|C  Length=0.1  Frequency=60  Resistances=[ 0.01273 0.3864]  Inductances="[ 0.9337e-3  4.1264e-3]"  Capacitances=[12.74e-9 7.751e-9]
  line30_2 : powerlib/Elements/Three-Phase PI Section Line  LConnTagsString=a|b|c  RConnTagsString=A|B|C  Length=0.9  Frequency=60  Resistances=[ 0.01273 0.3864]  Inductances="[ 0.9337e-3  4.1264e-3]"  Capacitances=[12.74e-9 7.751e-9]
  line31_1 : powerlib/Elements/Three-Phase PI Section Line  LConnTagsString=a|b|c  RConnTagsString=A|B|C  Length=0.1  Frequency=60  Resistances=[ 0.01273 0.3864]  Inductances="[ 0.9337e-3  4.1264e-3]"  Capacitances=[12.74e-9 7.751e-9]
  line31_2 : powerlib/Elements/Three-Phase PI Section Line  LConnTagsString=a|b|c  RConnTagsString=A|B|C  Length=0.9  Frequency=60  Resistances=[ 0.01273 0.3864]  Inductances="[ 0.9337e-3  4.1264e-3]"  Capacitances=[12.74e-9 7.751e-9]
  line32_1 : powerlib/Elements/Three-Phase PI Section Line  LConnTagsString=a|b|c  RConnTagsString=A|B|C  Length=0.1  Frequency=60  Resistances=[ 0.01273 0.3864]  Inductances="[ 0.9337e-3  4.1264e-3]"  Capacitances=[12.74e-9 7.751e-9]
  line32_2 : powerlib/Elements/Three-Phase PI Section Line  LConnTagsString=a|b|c  RConnTagsString=A|B|C  Length=0.9  Frequency=60  Resistances=[ 0.01273 0.3864]  Inductances="[ 0.9337e-3  4.1264e-3]"  Capacitances=[12.74e-9 7.751e-9]
  line3_1 : powerlib/Elements/Three-Phase PI Section Line  LConnTagsString=a|b|c  RConnTagsString=A|B|C  Length=0.1  Frequency=60  Resistances=[ 0.01273 0.3864]  Inductances="[ 0.9337e-3  4.1264e-3]"  Capacitances=[12.74e-9 7.751e-9]
  line3_2 : powerlib/Elements/Three-Phase PI Section Line  LConnTagsString=a|b|c  RConnTagsString=A|B|C  Length=0.9  Frequency=60  Resistances=[ 0.01273 0.3864]  Inductances="[ 0.9337e-3  4.1264e-3]"  Capacitances=[12.74e-9 7.751e-9]
  line4_1 : powerlib/Elements/Three-Phase PI Section Line  LConnTagsString=a|b|c  RConnTagsString=A|B|C  Length=0.1  Frequency=60  Resistances=[ 0.01273 0.3864]  Inductances="[ 0.9337e-3  4.1264e-3]"  Capacitances=[12.74e-9 7.751e-9]
  line4_2 : powerlib/Elements/Three-Phase PI Section Line  LConnTagsString=a|b|c  RConnTagsString=A|B|C  Length=0.9  Frequency=60  Resistances=[ 0.01273 0.3864]  Inductances="[ 0.9337e-3  4.1264e-3]"  Capacitances=[12.74e-9 7.751e-9]
  line5_1 : powerlib/Elements/Three-Phase PI Section Line  LConnTagsString=a|b|c  RConnTagsString=A|B|C  Length=0.1  Frequency=60  Resistances=[ 0.01273 0.3864]  Inductances="[ 0.9337e-3  4.1264e-3]"  Capacitances=[12.74e-9 7.751e-9]
  line5_2 : powerlib/Elements/Three-Phase PI Section Line  LConnTagsString=a|b|c  RConnTagsString=A|B|C  Length=0.9  Frequency=60  Resistances=[ 0.01273 0.3864]  Inductances="[ 0.9337e-3  4.1264e-3]"  Capacitances=[12.74e-9 7.751e-9]
  line6_1 : powerlib/Elements/Three-Phase PI Section Line  LConnTagsString=a|b|c  RConnTagsString=A|B|C  Length=0.1  Frequency=60  Resistances=[ 0.01273 0.3864]  Inductances="[ 0.9337e-3  4.1264e-3]"  Capacitances=[12.74e-9 7.751e-9]
  line6_2 : powerlib/Elements/Three-Phase PI Section Line  LConnTagsString=a|b|c  RConnTagsString=A|B|C  Length=0.9  Frequency=60  Resistances=[ 0.01273 0.3864]  Inductances="[ 0.9337e-3  4.1264e-3]"  Capacitances=[12.74e-9 7.751e-9]
  line7_1 : powerlib/Elements/Three-Phase PI Section Line  LConnTagsString=a|b|c  RConnTagsString=A|B|C  Length=0.1  Frequency=60  Resistances=[ 0.01273 0.3864]  Inductances="[ 0.9337e-3  4.1264e-3]"  Capacitances=[12.74e-9 7.751e-9]
  line7_2 : powerlib/Elements/Three-Phase PI Section Line  LConnTagsString=a|b|c  RConnTagsString=A|B|C  Length=0.9  Frequency=60  Resistances=[ 0.01273 0.3864]  Inductances="[ 0.9337e-3  4.1264e-3]"  Capacitances=[12.74e-9 7.751e-9]
  line8_1 : powerlib/Elements/Three-Phase PI Section Line  LConnTagsString=a|b|c  RConnTagsString=A|B|C  Length=0.1  Frequency=60  Resistances=[ 0.01273 0.3864]  Inductances="[ 0.9337e-3  4.1264e-3]"  Capacitances=[12.74e-9 7.751e-9]
  line8_2 : powerlib/Elements/Three-Phase PI Section Line  LConnTagsString=a|b|c  RConnTagsString=A|B|C  Length=0.9  Frequency=60  Resistances=[ 0.01273 0.3864]  Inductances="[ 0.9337e-3  4.1264e-3]"  Capacitances=[12.74e-9 7.751e-9]
  line9_1 : powerlib/Elements/Three-Phase PI Section Line  LConnTagsString=a|b|c  RConnTagsString=A|B|C  Length=0.1  Frequency=60  Resistances=[ 0.01273 0.3864]  Inductances="[ 0.9337e-3  4.1264e-3]"  Capacitances=[12.74e-9 7.751e-9]
  line9_2 : powerlib/Elements/Three-Phase PI Section Line  LConnTagsString=a|b|c  RConnTagsString=A|B|C  Length=0.9  Frequency=60  Resistances=[ 0.01273 0.3864]  Inductances="[ 0.9337e-3  4.1264e-3]"  Capacitances=[12.74e-9 7.751e-9]
  powergui : powerlib/powergui  Priority=1  SimulationMode=Discrete  SampleTime=50e-6  frequency=60  Iterations=50  frequencyindice=50  Pbase=100e6  ErrMax=1e-4  UnitsV=kV  UnitsW=MW  buscounter=0  FunctionMessages=off  echomessages=off  EnableUseOfTLC=off  CurrentSourceSwitches=off  DisableSnubberDevices=off  DisableRonSwitches=off  DisableVfSwitches=off  DisplayEquations=off  AutomaticDiscreteSolvers=off  SolverType=Tustin/Backward Euler (TBE)  Interpol=off  ExternalGateDelay=off  methode=off  Ts=100  x0status=blocks  SPID=on  SwTol=0  HookPort=off  NonlinearTolerance=1e-4  nMaxIteration=100  ContinueOnMaxIteration=off  RestoreLinks=warning  ResistiveCurrentMeasurement=off  Frange=[0:2:500]  Ylog=off  Xlog=on  ShowGrid=off  save=off  variable=ZData  structure=0  ZoomFFT=off  StartTime=0.0  cycles=1  DisplayStyle=1  fundamental=60  FreqAxis=off  MaxFrequency=1000  frequencyindicesteady=1  RmsSteady=1  display=off
  wires:
  Three-Phase V-I Measurement21/1 -> Scope/1
  Three-Phase V-I Measurement21/2 -> Scope1/1
  connections:
  line1_2/LConn2 -- line1_1/RConn2
  line1_2/LConn3 -- line1_1/RConn3
  line1_1/RConn1 -- line1_2/LConn1
  line1_1/LConn1 -- Three-Phase V-I Measurement/RConn1
  Three-Phase Transformer (Two Windings)/LConn4 -- Ground/LConn1
  Three-Phase Transformer (Two Windings)/RConn3 -- Three-Phase V-I Measurement/LConn3
  Three-Phase Transformer (Two Windings)/LConn2 -- Three-Phase Source/RConn2
  Three-Phase Transformer (Two Windings)/RConn1 -- Three-Phase V-I Measurement/LConn1
  Three-Phase Source/RConn3 -- Three-Phase Transformer (Two Windings)/LConn3
  Three-Phase Transformer (Two Windings)/RConn2 -- Three-Phase V-I Measurement/LConn2
  line1_1/LConn3 -- Three-Phase V-I Measurement/RConn3
  Three-Phase Source/RConn1 -- Three-Phase Transformer (Two Windings)/LConn1
  line1_2/RConn2 -- Three-Phase V-I Measurement1/LConn2
  line1_2/RConn3 -- Three-Phase V-I Measurement1/LConn3
  line1_2/RConn1 -- Three-Phase V-I Measurement1/LConn1
  line1_1/LConn2 -- Three-Phase V-I Measurement/RConn2
  Three-Phase V-I Measurement1/RConn2 -- line18_1/LConn2 -- line2_1/LConn2 -- Node1/LConn2
  Three-Phase V-I Measurement1/RConn1 -- line18_1/LConn1 -- line2_1/LConn1 -- Node1/LConn1
  Three-Phase V-I Measurement1/RConn3 -- Node1/LConn3 -- line18_1/LConn3 -- line2_1/LConn3
  line2_1/RConn1 -- line2_2/LConn1
  Three-Phase V-I Measurement2/LConn1 -- line2_2/RConn1
  Three-Phase V-I Measurement2/LConn2 -- line2_2/RConn2
  Three-Phase V-I Measurement2/LConn3 -- line2_2/RConn3
  line2_2/LConn3 -- line2_1/RConn3
  line2_2/LConn2 -- line2_1/RConn2
  Node2/LConn3 -- line22_1/LConn3 -- line3_1/LConn3 -- Three-Phase V-I Measurement2/RConn3
  Node2/LConn2 -- line22_1/LConn2 -- line3_1/LConn2 -- Three-Phase V-I Measurement2/RConn2
  Node2/LConn1 -- line22_1/LConn1 -- line3_1/LConn1 -- Three-Phase V-I Measurement2/RConn1
  Node3/LConn1 -- line4_1/LConn1 -- Three-Phase V-I Measurement3/RConn1
  Node3/LConn2 -- Three-Phase V-I Measurement3/RConn2 -- line4_1/LConn2
  Node3/LConn3 -- Three-Phase V-I Measurement3/RConn3 -- line4_1/LConn3
  Three-Phase V-I Measurement3/LConn3 -- line3_2/RConn3
  Three-Phase V-I Measurement3/LConn1 -- line3_2/RConn1
  line3_2/LConn3 -- line3_1/RConn3
  Three-Phase V-I Measurement3/LConn2 -- line3_2/RConn2
  line3_2/LConn2 -- line3_1/RConn2
  line3_1/RConn1 -- line3_2/LConn1
  Node4/LConn1 -- line5_1/LConn1 -- Three-Phase V-I Measurement4/RConn1
  Node4/LConn2 -- line5_1/LConn2 -- Three-Phase V-I Measurement4/RConn2
  Node4/LConn3 -- line5_1/LConn3 -- Three-Phase V-I Measurement4/RConn3
  Three-Phase V-I Measurement4/LConn3 -- line4_2/RConn3
  Three-Phase V-I Measurement4/LConn1 -- line4_2/RConn1
  line4_2/LConn3 -- line4_1/RConn3
  Three-Phase V-I Measurement4/LConn2 -- line4_2/RConn2
  line4_2/LConn2 -- line4_1/RConn2
  line4_1/RConn1 -- line4_2/LConn1
  Node5/LConn1 -- line25_1/LConn1 -- line6_1/LConn1 -- Three-Phase V-I Measurement5/RConn1
  Node5/LConn2 -- line25_1/LConn2 -- line6_1/LConn2 -- Three-Phase V-I Measurement5/RConn2
  Node5/LConn3 -- line25_1/LConn3 -- line6_1/LConn3 -- Three-Phase V-I Measurement5/RConn3
  Three-Phase V-I Measurement5/LConn3 -- line5_2/RConn3
  Three-Phase V-I Measurement5/LConn1 -- line5_2/RConn1
  line5_2/LConn3 -- line5_1/RConn3
  Three-Phase V-I Measurement5/LConn2 -- line5_2/RConn2
  line5_2/LConn2 -- line5_1/RConn2
  line5_1/RConn1 -- line5_2/LConn1
  Node6/LConn2 -- line7_1/LConn2 -- Three-Phase V-I Measurement6/RConn2
  Node6/LConn1 -- line7_1/LConn1 -- Three-Phase V-I Measurement6/RConn1
  Node6/LConn3 -- line7_1/LConn3 -- Three-Phase V-I Measurement6/RConn3
  line6_2/LConn3 -- line6_1/RConn3
  line6_1/RConn1 -- line6_2/LConn1
  Three-Phase V-I Measurement6/LConn2 -- line6_2/RConn2
  line6_2/LConn2 -- line6_1/RConn2
  Three-Phase V-I Measurement6/LConn3 -- line6_2/RConn3
  Three-Phase V-I Measurement6/LConn1 -- line6_2/RConn1
  Node7/LConn2 -- line8_1/LConn2 -- Three-Phase V-I Measurement7/RConn2
  Node7/LConn1 -- line8_1/LConn1 -- Three-Phase V-I Measurement7/RConn1
  Node7/LConn3 -- line8_1/LConn3 -- Three-Phase V-I Measurement7/RConn3
  line7_2/LConn3 -- line7_1/RConn3
  line7_1/RConn1 -- line7_2/LConn1
  Three-Phase V-I Measurement7/LConn2 -- line7_2/RConn2
  line7_2/LConn2 -- line7_1/RConn2
  Three-Phase V-I Measurement7/LConn3 -- line7_2/RConn3
  Three-Phase V-I Measurement7/LConn1 -- line7_2/RConn1
  Node8/LConn2 -- line9_1/LConn2 -- Three-Phase V-I Measurement8/RConn2
  Node8/LConn1 -- line9_1/LConn1 -- Three-Phase V-I Measurement8/RConn1
  Node8/LConn3 -- line9_1/LConn3 -- Three-Phase V-I Measurement8/RConn3
  line8_2/LConn3 -- line8_1/RConn3
  line8_1/RConn1 -- line8_2/LConn1
  Three-Phase V-I Measurement8/LConn2 -- line8_2/RConn2
  line8_2/LConn2 -- line8_1/RConn2
  Three-Phase V-I Measurement8/LConn3 -- line8_2/RConn3
  Three-Phase V-I Measurement8/LConn1 -- line8_2/RConn1
  Node12/LConn3 -- line13_1/LConn3 -- Three-Phase V-I Measurement12/RConn3
  Node9/LConn2 -- line10_1/LConn2 -- Three-Phase V-I Measurement9/RConn2
  Node9/LConn3 -- line10_1/LConn3 -- Three-Phase V-I Measurement9/RConn3
  Node12/LConn2 -- line13_1/LConn2 -- Three-Phase V-I Measurement12/RConn2
  Node13/LConn3 -- line14_1/LConn3 -- Three-Phase V-I Measurement13/RConn3
  Node10/LConn2 -- line11_1/LConn2 -- Three-Phase V-I Measurement10/RConn2
  Node10/LConn1 -- line11_1/LConn1 -- Three-Phase V-I Measurement10/RConn1
  Node10/LConn3 -- line11_1/LConn3 -- Three-Phase V-I Measurement10/RConn3
  Node13/LConn1 -- line14_1/LConn1 -- Three-Phase V-I Measurement13/RConn1
  Node9/LConn1 -- line10_1/LConn1 -- Three-Phase V-I Measurement9/RConn1
  Node11/LConn1 -- line12_1/LConn1 -- Three-Phase V-I Measurement11/RConn1
  Node12/LConn1 -- line13_1/LConn1 -- Three-Phase V-I Measurement12/RConn1
  Node13/LConn2 -- line14_1/LConn2 -- Three-Phase V-I Measurement13/RConn2
  Node11/LConn3 -- line12_1/LConn3 -- Three-Phase V-I Measurement11/RConn3
  Node11/LConn2 -- line12_1/LConn2 -- Three-Phase V-I Measurement11/RConn2
  line12_2/LConn2 -- line12_1/RConn2
  Three-Phase V-I Measurement12/LConn2 -- line12_2/RConn2
  Three-Phase V-I Measurement11/LConn1 -- line11_2/RConn1
  line10_2/LConn3 -- line10_1/RConn3
  line12_1/RConn1 -- line12_2/LConn1
  line9_2/LConn2 -- line9_1/RConn2
  line9_2/LConn3 -- line9_1/RConn3
  Three-Phase V-I Measurement9/LConn1 -- line9_2/RConn1
  line13_1/RConn1 -- line13_2/LConn1
  line9_1/RConn1 -- line9_2/LConn1
  line13_2/LConn2 -- line13_1/RConn2
  Three-Phase V-I Measurement11/LConn3 -- line11_2/RConn3
  line10_2/LConn2 -- line10_1/RConn2
  Three-Phase V-I Measurement12/LConn3 -- line12_2/RConn3
  Three-Phase V-I Measurement10/LConn2 -- line10_2/RConn2
  Three-Phase V-I Measurement12/LConn1 -- line12_2/RConn1
  Three-Phase V-I Measurement13/LConn3 -- line13_2/RConn3
  line11_1/RConn1 -- line11_2/LConn1
  line11_2/LConn3 -- line11_1/RConn3
  Three-Phase V-I Measurement13/LConn2 -- line13_2/RConn2
  Three-Phase V-I Measurement9/LConn3 -- line9_2/RConn3
  Three-Phase V-I Measurement10/LConn1 -- line10_2/RConn1
  line12_2/LConn3 -- line12_1/RConn3
  Three-Phase V-I Measurement11/LConn2 -- line11_2/RConn2
  Three-Phase V-I Measurement13/LConn1 -- line13_2/RConn1
  Three-Phase V-I Measurement9/LConn2 -- line9_2/RConn2
  Three-Phase V-I Measurement10/LConn3 -- line10_2/RConn3
  line11_2/LConn2 -- line11_1/RConn2
  line10_1/RConn1 -- line10_2/LConn1
  line13_2/LConn3 -- line13_1/RConn3
  Node16/LConn1 -- line17_1/LConn1 -- Three-Phase V-I Measurement16/RConn1
  Node14/LConn3 -- line15_1/LConn3 -- Three-Phase V-I Measurement14/RConn3
  Node15/LConn1 -- line16_1/LConn1 -- Three-Phase V-I Measurement15/RConn1
  Node14/LConn1 -- line15_1/LConn1 -- Three-Phase V-I Measurement14/RConn1
  Node15/LConn3 -- line16_1/LConn3 -- Three-Phase V-I Measurement15/RConn3
  Node15/LConn2 -- line16_1/LConn2 -- Three-Phase V-I Measurement15/RConn2
  Node14/LConn2 -- line15_1/LConn2 -- Three-Phase V-I Measurement14/RConn2
  Node16/LConn3 -- line17_1/LConn3 -- Three-Phase V-I Measurement16/RConn3
  Node16/LConn2 -- line17_1/LConn2 -- Three-Phase V-I Measurement16/RConn2
  line15_1/RConn1 -- line15_2/LConn1
  line14_1/RConn1 -- line14_2/LConn1
  line15_2/LConn2 -- line15_1/RConn2
  Three-Phase V-I Measurement17/LConn2 -- line17_2/RConn2
  Three-Phase V-I Measurement14/LConn3 -- line14_2/RConn3
  Three-Phase V-I Measurement16/LConn1 -- line16_2/RConn1
  line15_2/LConn3 -- line15_1/RConn3
  Three-Phase V-I Measurement14/LConn2 -- line14_2/RConn2
  line14_2/LConn3 -- line14_1/RConn3
  Three-Phase V-I Measurement15/LConn1 -- line15_2/RConn1
  Three-Phase V-I Measurement14/LConn1 -- line14_2/RConn1
  line17_1/RConn1 -- line17_2/LConn1
  line17_2/LConn3 -- line17_1/RConn3
  Three-Phase V-I Measurement17/LConn1 -- line17_2/RConn1
  line16_1/RConn1 -- line16_2/LConn1
  line14_2/LConn2 -- line14_1/RConn2
  Node17/LConn1 -- Three-Phase V-I Measurement17/RConn1
  Three-Phase V-I Measurement15/LConn3 -- line15_2/RConn3
  Node17/LConn3 -- Three-Phase V-I Measurement17/RConn3
  Three-Phase V-I Measurement16/LConn3 -- line16_2/RConn3
  Node17/LConn2 -- Three-Phase V-I Measurement17/RConn2
  Three-Phase V-I Measurement17/LConn3 -- line17_2/RConn3
  Three-Phase V-I Measurement16/LConn2 -- line16_2/RConn2
  Three-Phase V-I Measurement15/LConn2 -- line15_2/RConn2
  line16_2/LConn2 -- line16_1/RConn2
  line17_2/LConn2 -- line17_1/RConn2
  line16_2/LConn3 -- line16_1/RConn3
  Node20/LConn1 -- line21_1/LConn1 -- Three-Phase V-I Measurement20/RConn1
  Node18/LConn3 -- line19_1/LConn3 -- Three-Phase V-I Measurement18/RConn3
  Node19/LConn1 -- line20_1/LConn1 -- Three-Phase V-I Measurement19/RConn1
  Node18/LConn1 -- line19_1/LConn1 -- Three-Phase V-I Measurement18/RConn1
  Node19/LConn3 -- line20_1/LConn3 -- Three-Phase V-I Measurement19/RConn3
  Node19/LConn2 -- line20_1/LConn2 -- Three-Phase V-I Measurement19/RConn2
  Node18/LConn2 -- line19_1/LConn2 -- Three-Phase V-I Measurement18/RConn2
  Node20/LConn3 -- line21_1/LConn3 -- Three-Phase V-I Measurement20/RConn3
  Node20/LConn2 -- line21_1/LConn2 -- Three-Phase V-I Measurement20/RConn2
  line19_1/RConn1 -- line19_2/LConn1
  line18_1/RConn1 -- line18_2/LConn1
  line19_2/LConn2 -- line19_1/RConn2
  Three-Phase V-I Measurement21/LConn2 -- line21_2/RConn2
  Three-Phase V-I Measurement18/LConn3 -- line18_2/RConn3
  Three-Phase V-I Measurement20/LConn1 -- line20_2/RConn1
  line19_2/LConn3 -- line19_1/RConn3
  Three-Phase V-I Measurement18/LConn2 -- line18_2/RConn2
  line18_2/LConn3 -- line18_1/RConn3
  Three-Phase V-I Measurement19/LConn1 -- line19_2/RConn1
  Three-Phase V-I Measurement18/LConn1 -- line18_2/RConn1
  line21_1/RConn1 -- line21_2/LConn1
  line21_2/LConn3 -- line21_1/RConn3
  Three-Phase V-I Measurement21/LConn1 -- line21_2/RConn1
  line20_1/RConn1 -- line20_2/LConn1
  line18_2/LConn2 -- line18_1/RConn2
  Node21/LConn1 -- Three-Phase V-I Measurement21/RConn1
  Three-Phase V-I Measurement19/LConn3 -- line19_2/RConn3
  Node21/LConn3 -- Three-Phase V-I Measurement21/RConn3
  Three-Phase V-I Measurement20/LConn3 -- line20_2/RConn3
  Node21/LConn2 -- Three-Phase V-I Measurement21/RConn2
  Three-Phase V-I Measurement21/LConn3 -- line21_2/RConn3
  Three-Phase V-I Measurement20/LConn2 -- line20_2/RConn2
  Three-Phase V-I Measurement19/LConn2 -- line19_2/RConn2
  line20_2/LConn2 -- line20_1/RConn2
  line21_2/LConn2 -- line21_1/RConn2
  line20_2/LConn3 -- line20_1/RConn3
  Node22/LConn2 -- line23_1/LConn2 -- Three-Phase V-I Measurement22/RConn2
  Node23/LConn3 -- line24_1/LConn3 -- Three-Phase V-I Measurement23/RConn3
  Node23/LConn1 -- line24_1/LConn1 -- Three-Phase V-I Measurement23/RConn1
  Node22/LConn1 -- line23_1/LConn1 -- Three-Phase V-I Measurement22/RConn1
  Node22/LConn3 -- line23_1/LConn3 -- Three-Phase V-I Measurement22/RConn3
  Node23/LConn2 -- line24_1/LConn2 -- Three-Phase V-I Measurement23/RConn2
  line24_2/LConn3 -- line24_1/RConn3
  line22_2/LConn3 -- line22_1/RConn3
  Three-Phase V-I Measurement24/LConn1 -- line24_2/RConn1
  line23_2/LConn2 -- line23_1/RConn2
  line24_1/RConn1 -- line24_2/LConn1
  line23_2/LConn3 -- line23_1/RConn3
  Three-Phase V-I Measurement23/LConn3 -- line23_2/RConn3
  Node24/LConn3 -- Three-Phase V-I Measurement24/RConn3
  Three-Phase V-I Measurement22/LConn3 -- line22_2/RConn3
  line24_2/LConn2 -- line24_1/RConn2
  Node24/LConn1 -- Three-Phase V-I Measurement24/RConn1
  Three-Phase V-I Measurement24/LConn3 -- line24_2/RConn3
  Node24/LConn2 -- Three-Phase V-I Measurement24/RConn2
  line22_1/RConn1 -- line22_2/LConn1
  Three-Phase V-I Measurement24/LConn2 -- line24_2/RConn2
  Three-Phase V-I Measurement23/LConn2 -- line23_2/RConn2
  Three-Phase V-I Measurement23/LConn1 -- line23_2/RConn1
  Three-Phase V-I Measurement22/LConn1 -- line22_2/RConn1
  line22_2/LConn2 -- line22_1/RConn2
  Three-Phase V-I Measurement22/LConn2 -- line22_2/RConn2
  line23_1/RConn1 -- line23_2/LConn1
  Three-Phase V-I Measurement28/RConn2 -- Node28/LConn2 -- line29_1/LConn2
  Node26/LConn3 -- line27_1/LConn3 -- Three-Phase V-I Measurement26/RConn3
  Node27/LConn1 -- line28_1/LConn1 -- Three-Phase V-I Measurement27/RConn1
  Node31/LConn3 -- line32_1/LConn3 -- Three-Phase V-I Measurement31/RConn3
  Node25/LConn3 -- line26_1/LConn3 -- Three-Phase V-I Measurement25/RConn3
  Node30/LConn3 -- line31_1/LConn3 -- Three-Phase V-I Measurement30/RConn3
  Node29/LConn2 -- line30_1/LConn2 -- Three-Phase V-I Measurement29/RConn2
  Node31/LConn1 -- line32_1/LConn1 -- Three-Phase V-I Measurement31/RConn1
  Node25/LConn2 -- line26_1/LConn2 -- Three-Phase V-I Measurement25/RConn2
  Node26/LConn1 -- line27_1/LConn1 -- Three-Phase V-I Measurement26/RConn1
  Node29/LConn3 -- line30_1/LConn3 -- Three-Phase V-I Measurement29/RConn3
  Node30/LConn1 -- line31_1/LConn1 -- Three-Phase V-I Measurement30/RConn1
  Three-Phase V-I Measurement28/RConn1 -- line29_1/LConn1 -- Node28/LConn1
  Node27/LConn2 -- line28_1/LConn2 -- Three-Phase V-I Measurement27/RConn2
  Node31/LConn2 -- line32_1/LConn2 -- Three-Phase V-I Measurement31/RConn2
  Node27/LConn3 -- line28_1/LConn3 -- Three-Phase V-I Measurement27/RConn3
  Node26/LConn2 -- line27_1/LConn2 -- Three-Phase V-I Measurement26/RConn2
  Node30/LConn2 -- line31_1/LConn2 -- Three-Phase V-I Measurement30/RConn2
  Node25/LConn1 -- line26_1/LConn1 -- Three-Phase V-I Measurement25/RConn1
  Three-Phase V-I Measurement28/RConn3 -- Node28/LConn3 -- line29_1/LConn3
  Node29/LConn1 -- line30_1/LConn1 -- Three-Phase V-I Measurement29/RConn1
  line30_2/LConn2 -- line30_1/RConn2
  Three-Phase V-I Measurement27/LConn3 -- line27_2/RConn3
  line27_2/LConn3 -- line27_1/RConn3
  Three-Phase V-I Measurement29/LConn3 -- line29_2/RConn3
  line28_2/LConn3 -- line28_1/RConn3
  line26_2/LConn2 -- line26_1/RConn2
  line27_1/RConn1 -- line27_2/LConn1
  Three-Phase V-I Measurement28/LConn1 -- line28_2/RConn1
  line25_1/RConn1 -- line25_2/LConn1
  line29_1/RConn1 -- line29_2/LConn1
  Three-Phase V-I Measurement25/LConn1 -- line25_2/RConn1
  Three-Phase V-I Measurement26/LConn3 -- line26_2/RConn3
  Three-Phase V-I Measurement27/LConn1 -- line27_2/RConn1
  Three-Phase V-I Measurement27/LConn2 -- line27_2/RConn2
  line26_2/LConn3 -- line26_1/RConn3
  line30_1/RConn1 -- line30_2/LConn1
  line25_2/LConn2 -- line25_1/RConn2
  line27_2/LConn2 -- line27_1/RConn2
  line29_2/LConn2 -- line29_1/RConn2
  line28_2/LConn2 -- line28_1/RConn2
  Three-Phase V-I Measurement31/LConn3 -- line31_2/RConn3
  Node32/LConn3 -- Three-Phase V-I Measurement32/RConn3
  Node32/LConn1 -- Three-Phase V-I Measurement32/RConn1
  line31_1/RConn1 -- line31_2/LConn1
  Node32/LConn2 -- Three-Phase V-I Measurement32/RConn2
  Three-Phase V-I Measurement25/LConn3 -- line25_2/RConn3
  Three-Phase V-I Measurement28/LConn3 -- line28_2/RConn3
  Three-Phase V-I Measurement29/LConn2 -- line29_2/RConn2
  Three-Phase V-I Measurement30/LConn3 -- line30_2/RConn3
  Three-Phase V-I Measurement28/LConn2 -- line28_2/RConn2
  Three-Phase V-I Measurement26/LConn2 -- line26_2/RConn2
  line26_1/RConn1 -- line26_2/LConn1
  Three-Phase V-I Measurement26/LConn1 -- line26_2/RConn1
  Three-Phase V-I Measurement31/LConn2 -- line31_2/RConn2
  Three-Phase V-I Measurement30/LConn2 -- line30_2/RConn2
  line31_2/LConn2 -- line31_1/RConn2
  line25_2/LConn3 -- line25_1/RConn3
  Three-Phase V-I Measurement31/LConn1 -- line31_2/RConn1
  line32_1/RConn1 -- line32_2/LConn1
  Three-Phase V-I Measurement25/LConn2 -- line25_2/RConn2
  line28_1/RConn1 -- line28_2/LConn1
  line32_2/LConn3 -- line32_1/RConn3
  Three-Phase V-I Measurement30/LConn1 -- line30_2/RConn1
  line32_2/LConn2 -- line32_1/RConn2
  line29_2/LConn3 -- line29_1/RConn3
  Three-Phase V-I Measurement29/LConn1 -- line29_2/RConn1
  Three-Phase V-I Measurement32/LConn1 -- line32_2/RConn1
  line30_2/LConn3 -- line30_1/RConn3
  line31_2/LConn3 -- line31_1/RConn3
  Three-Phase V-I Measurement32/LConn2 -- line32_2/RConn2
  Three-Phase V-I Measurement32/LConn3 -- line32_2/RConn3
